simulink model "s_b2a4x1kf"  (R2018b)
settings: Solver=VariableStepDiscrete  StartTime=0.0  StopTime=100  RelTol=1e-3
undefined symbols (not defined in the file): fft_stages, n_bits_ants, n_bits_xengs
libraries: xbsIndex_r4 x20671, casper_library_misc x69, casper_library_scopes x15, casper_library_delays x8, xbsReplacements_r4 x6, xps_library x4
(part 2 of 212)

== system s_b2a4x1kf/Delay10 ==
  d : Inport
  Register0 : xbsIndex_r4/Register  init=0  rst=off  en=off  dbl_ovrd=off  block_type=register
      settings: block_version=11.4
  Register1 : xbsIndex_r4/Register  init=0  rst=off  en=off  dbl_ovrd=off  block_type=register
      settings: block_version=11.4
  q : Outport
  wires:
  Register0/1 -> Register1/1
  d/1 -> Register0/1
  Register1/1 -> q/1

== system s_b2a4x1kf/Delay16 ==
  d : Inport
  Register0 : xbsIndex_r4/Register  init=0  rst=off  en=off  dbl_ovrd=off  block_type=register
      settings: block_version=11.4
  Register1 : xbsIndex_r4/Register  init=0  rst=off  en=off  dbl_ovrd=off  block_type=register
      settings: block_version=11.4
  q : Outport
  wires:
  Register0/1 -> Register1/1
  d/1 -> Register0/1
  Register1/1 -> q/1

== system s_b2a4x1kf/Delay18 ==
  d : Inport
  Register0 : xbsIndex_r4/Register  init=0  rst=off  en=off  dbl_ovrd=off  block_type=register
      settings: block_version=11.4
  Register1 : xbsIndex_r4/Register  init=0  rst=off  en=off  dbl_ovrd=off  block_type=register
      settings: block_version=11.4
  q : Outport
  wires:
  Register0/1 -> Register1/1
  d/1 -> Register0/1
  Register1/1 -> q/1

== system s_b2a4x1kf/Delay19 ==
  d : Inport
  Register0 : xbsIndex_r4/Register  init=0  rst=off  en=off  dbl_ovrd=off  block_type=register
      settings: block_version=11.4
  Register1 : xbsIndex_r4/Register  init=0  rst=off  en=off  dbl_ovrd=off  block_type=register
      settings: block_version=11.4
  q : Outport
  wires:
  Register0/1 -> Register1/1
  d/1 -> Register0/1
  Register1/1 -> q/1

== system s_b2a4x1kf/Delay20 ==
  d : Inport
  Register0 : xbsIndex_r4/Register  init=0  rst=off  en=off  dbl_ovrd=off  block_type=register
      settings: block_version=11.4
  Register1 : xbsIndex_r4/Register  init=0  rst=off  en=off  dbl_ovrd=off  block_type=register
      settings: block_version=11.4
  q : Outport
  wires:
  Register0/1 -> Register1/1
  d/1 -> Register0/1
  Register1/1 -> q/1

== system s_b2a4x1kf/Delay21 ==
  d : Inport
  Register0 : xbsIndex_r4/Register  init=0  rst=off  en=off  dbl_ovrd=off  block_type=register
      settings: block_version=11.4
  Register1 : xbsIndex_r4/Register  init=0  rst=off  en=off  dbl_ovrd=off  block_type=register
      settings: block_version=11.4
  q : Outport
  wires:
  Register0/1 -> Register1/1
  d/1 -> Register0/1
  Register1/1 -> q/1

== system s_b2a4x1kf/Delay26 ==
  d : Inport
  Register0 : xbsIndex_r4/Register  init=0  rst=off  en=off  dbl_ovrd=off  block_type=register
      settings: block_version=11.4
  Register1 : xbsIndex_r4/Register  init=0  rst=off  en=off  dbl_ovrd=off  block_type=register
      settings: block_version=11.4
  q : Outport
  wires:
  Register0/1 -> Register1/1
  d/1 -> Register0/1
  Register1/1 -> q/1

== system s_b2a4x1kf/Delay27 ==
  d : Inport
  Register0 : xbsIndex_r4/Register  init=0  rst=off  en=off  dbl_ovrd=off  block_type=register
      settings: block_version=11.4
  Register1 : xbsIndex_r4/Register  init=0  rst=off  en=off  dbl_ovrd=off  block_type=register
      settings: block_version=11.4
  q : Outport
  wires:
  Register0/1 -> Register1/1
  d/1 -> Register0/1
  Register1/1 -> q/1

== system s_b2a4x1kf/Delay28 ==
  d : Inport
  Register0 : xbsIndex_r4/Register  init=0  rst=off  en=off  dbl_ovrd=off  block_type=register
      settings: block_version=11.4
  Register1 : xbsIndex_r4/Register  init=0  rst=off  en=off  dbl_ovrd=off  block_type=register
      settings: block_version=11.4
  q : Outport
  wires:
  Register0/1 -> Register1/1
  d/1 -> Register0/1
  Register1/1 -> q/1

== system s_b2a4x1kf/Delay32 ==
  d : Inport
  Register0 : xbsIndex_r4/Register  init=0  rst=off  en=off  dbl_ovrd=off  block_type=register
      settings: block_version=11.4
  Register1 : xbsIndex_r4/Register  init=0  rst=off  en=off  dbl_ovrd=off  block_type=register
      settings: block_version=11.4
  q : Outport
  wires:
  Register0/1 -> Register1/1
  d/1 -> Register0/1
  Register1/1 -> q/1

== system s_b2a4x1kf/Delay72 ==
  d : Inport
  Register0 : xbsIndex_r4/Register  init=0  rst=off  en=off  dbl_ovrd=off  block_type=register
      settings: block_version=11.4
  Register1 : xbsIndex_r4/Register  init=0  rst=off  en=off  dbl_ovrd=off  block_type=register
      settings: block_version=11.4
  q : Outport
  wires:
  Register0/1 -> Register1/1
  d/1 -> Register0/1
  Register1/1 -> q/1

== system s_b2a4x1kf/Delay9 ==
  d : Inport
  Register0 : xbsIndex_r4/Register  init=0  rst=off  en=off  dbl_ovrd=off  block_type=register
      settings: block_version=11.4
  Register1 : xbsIndex_r4/Register  init=0  rst=off  en=off  dbl_ovrd=off  block_type=register
      settings: block_version=11.4
  q : Outport
  wires:
  Register0/1 -> Register1/1
  d/1 -> Register0/1
  Register1/1 -> q/1

== system s_b2a4x1kf/Subsystem11 ==
  rst : Inport
  eof : Inport  Port=2
  valid : Inport  Port=3
  Counter11 : xbsIndex_r4/Counter  cnt_type=Free Running  cnt_to=Inf  operation=Up  start_count=0  cnt_by_val=1  arith_type=Unsigned  n_bits=n_bits_count  bin_pt=0  load_pin=off  rst=on  en=on  explicit_period=on  period=1  use_behavioral_HDL=off  implementation=Fabric  dbl_ovrd=off  block_type=counter
  Delay : xbsIndex_r4/Delay  rst=off  infoeditControl=Selection of Reset will increase slice count due to use of real FFs and instead of SRLs  en=off  latency=1  reg_retiming=on  dbl_ovrd=off  block_type=delay
      settings: infoedit=Hardware notes: A delay line is a chain, each link of which is an SRL16 or SRL32 followed by a flip-flop.
  Delay1 : xbsIndex_r4/Delay  rst=off  infoeditControl=Selection of Reset will increase slice count due to use of real FFs and instead of SRLs  en=off  latency=1  reg_retiming=on  dbl_ovrd=off  block_type=delay
      settings: infoedit=Hardware notes: A delay line is a chain, each link of which is an SRL16 or SRL32 followed by a flip-flop.
  Delay2 : xbsIndex_r4/Delay  rst=off  infoeditControl=Selection of Reset will increase slice count due to use of real FFs and instead of SRLs  en=off  latency=1  reg_retiming=on  dbl_ovrd=off  block_type=delay
      settings: infoedit=Hardware notes: A delay line is a chain, each link of which is an SRL16 or SRL32 followed by a flip-flop.
  Logical6 : xbsIndex_r4/Logical  logical_function=AND  inputs=2  en=off  latency=0  precision=Full  arith_type=Unsigned  n_bits=16  bin_pt=0  align_bp=on  dbl_ovrd=off  block_type=logical
  pipeline : Subsystem  Tag=cmac_delinked  mask(pipeline){csp_latency=2}
      mask prompts: csp_latency "Latency"
      mask help:
      | An explicitly laid-out delay line to avoid mapping to SRL16s
      | for use in pipelining to help achieve timing closure.
      mask init:
      | pipeline_init(gcb,'latency',csp_latency);
      settings: AttributesFormatString=Latency = %<latency>
      mask Display:
      | port_label('input', 1, 'd');
      | port_label('output', 1, 'q');
      | disp(['Z^-', num2str(csp_latency)]);
  out0 : Outport
  wires:
  pipeline/1(q) -> out0/1
  eof/1 -> Delay1/1
  Logical6/1 -> Counter11/2
  rst/1 -> Delay/1
  Delay/1 -> Counter11/1
  Counter11/1 -> pipeline/1(d)
  valid/1 -> Delay2/1
  Delay1/1 -> Logical6/1
  Delay2/1 -> Logical6/2

== system s_b2a4x1kf/Subsystem2 ==
  rst : Inport
  in0 : Inport  Port=2
  in1 : Inport  Port=3
  in2 : Inport  Port=4
  in3 : Inport  Port=5
  Counter{1..3,11} (4 alike) : xbsIndex_r4/Counter  cnt_type=Free Running  cnt_to=Inf  operation=Up  start_count=0  cnt_by_val=1  arith_type=Unsigned  n_bits=n_bits_count  bin_pt=0  load_pin=off  rst=on  en=on  explicit_period=on  period=1  use_behavioral_HDL=off  implementation=Fabric  dbl_ovrd=off  block_type=counter
  Delay{,1..4,15,17,59,61..63,76} (12 alike) : xbsIndex_r4/Delay  rst=off  infoeditControl=Selection of Reset will increase slice count due to use of real FFs and instead of SRLs  en=off  latency=1  reg_retiming=on  dbl_ovrd=off  block_type=delay
      settings: infoedit=Hardware notes: A delay line is a chain, each link of which is an SRL16 or SRL32 followed by a flip-flop.
  pipeline : Subsystem  Tag=cmac_delinked  mask(pipeline){csp_latency=2}
      mask prompts: csp_latency "Latency"
      mask help:
      | An explicitly laid-out delay line to avoid mapping to SRL16s
      | for use in pipelining to help achieve timing closure.
      mask init:
      | pipeline_init(gcb,'latency',csp_latency);
      settings: AttributesFormatString=Latency = %<latency>
      mask Display:
      | port_label('input', 1, 'd');
      | port_label('output', 1, 'q');
      | disp(['Z^-', num2str(csp_latency)]);
  pipeline1 : Subsystem  Tag=cmac_delinked  mask(pipeline){csp_latency=2}
      mask prompts: csp_latency "Latency"
      mask help:
      | An explicitly laid-out delay line to avoid mapping to SRL16s
      | for use in pipelining to help achieve timing closure.
      mask init:
      | pipeline_init(gcb,'latency',csp_latency);
      settings: AttributesFormatString=Latency = %<latency>
      mask Display:
      | port_label('input', 1, 'd');
      | port_label('output', 1, 'q');
      | disp(['Z^-', num2str(csp_latency)]);
  pipeline2 : Subsystem  Tag=cmac_delinked  mask(pipeline){csp_latency=2}
      mask prompts: csp_latency "Latency"
      mask help:
      | An explicitly laid-out delay line to avoid mapping to SRL16s
      | for use in pipelining to help achieve timing closure.
      mask init:
      | pipeline_init(gcb,'latency',csp_latency);
      settings: AttributesFormatString=Latency = %<latency>
      mask Display:
      | port_label('input', 1, 'd');
      | port_label('output', 1, 'q');
      | disp(['Z^-', num2str(csp_latency)]);
  pipeline3 : Subsystem  Tag=cmac_delinked  mask(pipeline){csp_latency=2}
      mask prompts: csp_latency "Latency"
      mask help:
      | An explicitly laid-out delay line to avoid mapping to SRL16s
      | for use in pipelining to help achieve timing closure.
      mask init:
      | pipeline_init(gcb,'latency',csp_latency);
      settings: AttributesFormatString=Latency = %<latency>
      mask Display:
      | port_label('input', 1, 'd');
      | port_label('output', 1, 'q');
      | disp(['Z^-', num2str(csp_latency)]);
  out0 : Outport
  out1 : Outport  Port=2
  out2 : Outport  Port=3
  out3 : Outport  Port=4
  wires:
  Counter11/1 -> pipeline/1(d)
  Counter1/1 -> pipeline1/1(d)
  Counter3/1 -> pipeline2/1(d)
  Delay17/1 -> Delay63/1
  Delay3/1 -> Delay62/1
  Delay15/1 -> Delay61/1
  Delay/1 -> Delay76/1, Counter11/1
  rst/1 -> Delay/1
  Delay61/1 -> Counter11/2
  Delay62/1 -> Counter1/2
  Delay63/1 -> Counter3/2
  Delay76/1 -> Counter1/1, Delay59/1
  in0/1 -> Delay15/1
  in1/1 -> Delay3/1
  in2/1 -> Delay17/1
  pipeline/1(q) -> out0/1
  pipeline1/1(q) -> out1/1
  pipeline2/1(q) -> out2/1
  Counter2/1 -> pipeline3/1(d)
  Delay1/1 -> Delay4/1
  Delay4/1 -> Counter2/2
  Delay59/1 -> Delay2/1, Counter3/1
  in3/1 -> Delay1/1
  pipeline3/1(q) -> out3/1
  Delay2/1 -> Counter2/1

== system s_b2a4x1kf/Subsystem7 ==
  dv : Inport
  Constant8 : xbsIndex_r4/Constant  const=clk_rate  gui_display_data_type=Fixed-point  arith_type=Unsigned  n_bits=ceil(log2(clk_rate))  bin_pt=0  preci_type=Single  exp_width=8  frac_width=24  explicit_period=on  period=1  equ=P=C  opselect=C  inp2=PCIN>>17  opr=+  inp1=P  carry=CIN  dbl_ovrd=off  block_type=constant
      settings: block_version=11.4
  Counter1 : xbsIndex_r4/Counter  cnt_type=Count Limited  cnt_to=clk_rate  operation=Up  start_count=0  cnt_by_val=1  arith_type=Unsigned  n_bits=ceil(log2(clk_rate))  bin_pt=0  load_pin=off  rst=off  en=off  explicit_period=on  period=1  use_behavioral_HDL=off  implementation=Fabric  dbl_ovrd=off  block_type=counter
  Counter6 : xbsIndex_r4/Counter  cnt_type=Free Running  cnt_to=Inf  operation=Up  start_count=0  cnt_by_val=1  arith_type=Unsigned  n_bits=32  bin_pt=0  load_pin=off  rst=on  en=on  explicit_period=on  period=1  use_behavioral_HDL=off  implementation=Fabric  dbl_ovrd=off  block_type=counter
  Delay : xbsIndex_r4/Delay  rst=off  infoeditControl=Selection of Reset will increase slice count due to use of real FFs and instead of SRLs  en=on  latency=1  reg_retiming=on  dbl_ovrd=off  block_type=delay
      settings: infoedit=Hardware notes: A delay line is a chain, each link of which is an SRL16 or SRL32 followed by a flip-flop.
  Delay5 : xbsIndex_r4/Delay  rst=off  infoeditControl=Selection of Reset will increase slice count due to use of real FFs and instead of SRLs  en=off  latency=1  reg_retiming=on  dbl_ovrd=off  block_type=delay
      settings: infoedit=Hardware notes: A delay line is a chain, each link of which is an SRL16 or SRL32 followed by a flip-flop.
  Relational : xbsIndex_r4/Relational  mode=a=b  op_type=Bool  en=off  latency=1  dbl_ovrd=off  block_type=relational
  per_sec : Outport
  wires:
  Delay/1 -> per_sec/1
  Counter6/1 -> Delay/1
  dv/1 -> Delay5/1
  Relational/1 -> Delay/2, Counter6/1
  Counter1/1 -> Relational/1
  Delay5/1 -> Counter6/2
  Constant8/1 -> Relational/2

== system s_b2a4x1kf/acc_len ==
  convert1_1 : DataTypeConversion  OutDataTypeStr=fixdt('ufix32_En0')  LockScale=on
  convert2_1 : DataTypeConversion  OutDataTypeStr=fixdt('ufix32_En0')  ConvertRealWorld=Stored Integer (SI)  LockScale=on
  gain_1 : Gain
  io_delay : xbsIndex_r4/Delay  rst=off  infoeditControl=Selection of Reset will increase slice count due to use of real FFs and instead of SRLs  en=off  latency=0  reg_retiming=on  dbl_ovrd=off  block_type=delay
  reint1 : xbsIndex_r4/Reinterpret  force_arith_type=on  arith_type=Unsigned  force_bin_pt=on  bin_pt=0  block_type=reinterpret
  s_b2a4x1kf_acc_len_user_data_out : xbsIndex_r4/Gateway In  gui_display_data_type=Fixed-point  arith_type=Unsigned  n_bits=32  bin_pt=0  preci_type=Single  exp_width=8  frac_width=24  rows=1  columns=1  quantization="Round  (unbiased: +/- Inf)"  overflow=Saturate  period=1  UseAsADC=off  ADCChannel='1'  interface=None  automatic_assignment=on  address_offset=hex2dec('00')  intf_name=''  intf_description=''  default_value=0  timing_constraint=None  locs_specified=off  LOCs={}  io_standard={}  inherit_from_input=off  hdl_port=on  dbl_ovrd=off  block_type=gatewayin
  sim_1 : Constant  Value=0
  slice_reg : xbsIndex_r4/Slice  nbits=32  boolean_output=off  mode=Lower Bit Location + Width  bit1=0  base1=MSB of Input  bit0=0  base0=LSB of Input  dbl_ovrd=off  block_type=slice
  in_reg : Outport
  wires:
  s_b2a4x1kf_acc_len_user_data_out/1 -> io_delay/1
  sim_1/1 -> convert1_1/1
  convert1_1/1 -> convert2_1/1
  convert2_1/1 -> gain_1/1
  gain_1/1 -> s_b2a4x1kf_acc_len_user_data_out/1
  io_delay/1 -> slice_reg/1
  slice_reg/1 -> reint1/1
  reint1/1 -> in_reg/1

== system s_b2a4x1kf/bf0_config ==
  convert1_1 : DataTypeConversion  OutDataTypeStr=fixdt('ufix15_En8')  LockScale=on
  convert1_2 : DataTypeConversion  OutDataTypeStr=fixdt('ufix16_En0')  LockScale=on
  convert1_3 : DataTypeConversion  OutDataTypeStr=fixdt('ufix1_En0')  LockScale=on
  convert2_1 : DataTypeConversion  OutDataTypeStr=fixdt('ufix15_En0')  ConvertRealWorld=Stored Integer (SI)  LockScale=on
  convert2_2 : DataTypeConversion  OutDataTypeStr=fixdt('ufix16_En0')  ConvertRealWorld=Stored Integer (SI)  LockScale=on
  convert2_3 : DataTypeConversion  OutDataTypeStr=fixdt('ufix1_En0')  ConvertRealWorld=Stored Integer (SI)  LockScale=on
  gain_1 : Gain  Gain=131072
  gain_2 : Gain  Gain=2
  gain_3 : Gain
  io_delay : xbsIndex_r4/Delay  rst=off  infoeditControl=Selection of Reset will increase slice count due to use of real FFs and instead of SRLs  en=off  latency=0  reg_retiming=on  dbl_ovrd=off  block_type=delay
  reint1 : xbsIndex_r4/Reinterpret  force_arith_type=on  arith_type=Unsigned  force_bin_pt=on  bin_pt=8  block_type=reinterpret
  reint2 : xbsIndex_r4/Reinterpret  force_arith_type=on  arith_type=Unsigned  force_bin_pt=on  bin_pt=0  block_type=reinterpret
  s_b2a4x1kf_bf0_config_user_data_out : xbsIndex_r4/Gateway In  gui_display_data_type=Fixed-point  arith_type=Unsigned  n_bits=32  bin_pt=0  preci_type=Single  exp_width=8  frac_width=24  rows=1  columns=1  quantization="Round  (unbiased: +/- Inf)"  overflow=Saturate  period=1  UseAsADC=off  ADCChannel='1'  interface=None  automatic_assignment=on  address_offset=hex2dec('00')  intf_name=''  intf_description=''  default_value=0  timing_constraint=None  locs_specified=off  LOCs={}  io_standard={}  inherit_from_input=off  hdl_port=on  dbl_ovrd=off  block_type=gatewayin
  sim_1 : Constant  Value=0
  sim_2 : Constant  Value=0
  sim_3 : Constant  Value=0
  sim_add : Sum  Inputs=+++  OutDataTypeStr=uint32
  slice_port : xbsIndex_r4/Slice  nbits=16  boolean_output=off  mode=Lower Bit Location + Width  bit1=0  base1=MSB of Input  bit0=1  base0=LSB of Input  dbl_ovrd=off  block_type=slice
  slice_quant_gain : xbsIndex_r4/Slice  nbits=15  boolean_output=off  mode=Lower Bit Location + Width  bit1=0  base1=MSB of Input  bit0=17  base0=LSB of Input  dbl_ovrd=off  block_type=slice
  slice_txen : xbsIndex_r4/Slice  nbits=1  boolean_output=on  mode=Lower Bit Location + Width  bit1=0  base1=MSB of Input  bit0=0  base0=LSB of Input  dbl_ovrd=off  block_type=slice
  in_quant_gain : Outport
  in_port : Outport  Port=2
  in_txen : Outport  Port=3
  wires:
  s_b2a4x1kf_bf0_config_user_data_out/1 -> io_delay/1
  sim_add/1 -> s_b2a4x1kf_bf0_config_user_data_out/1
  sim_1/1 -> convert1_1/1
  convert1_1/1 -> convert2_1/1
  convert2_1/1 -> gain_1/1
  gain_1/1 -> sim_add/1
  io_delay/1 -> slice_quant_gain/1, slice_port/1, slice_txen/1
  slice_quant_gain/1 -> reint1/1
  reint1/1 -> in_quant_gain/1
  sim_2/1 -> convert1_2/1
  convert1_2/1 -> convert2_2/1
  convert2_2/1 -> gain_2/1
  gain_2/1 -> sim_add/2
  slice_port/1 -> reint2/1
  reint2/1 -> in_port/1
  sim_3/1 -> convert1_3/1
  convert1_3/1 -> convert2_3/1
  convert2_3/1 -> gain_3/1
  gain_3/1 -> sim_add/3
  slice_txen/1 -> in_txen/1

== system s_b2a4x1kf/bf0_ip ==
  convert1_1 : DataTypeConversion  OutDataTypeStr=fixdt('ufix32_En0')  LockScale=on
  convert2_1 : DataTypeConversion  OutDataTypeStr=fixdt('ufix32_En0')  ConvertRealWorld=Stored Integer (SI)  LockScale=on
  gain_1 : Gain
  io_delay : xbsIndex_r4/Delay  rst=off  infoeditControl=Selection of Reset will increase slice count due to use of real FFs and instead of SRLs  en=off  latency=0  reg_retiming=on  dbl_ovrd=off  block_type=delay
  reint1 : xbsIndex_r4/Reinterpret  force_arith_type=on  arith_type=Unsigned  force_bin_pt=on  bin_pt=0  block_type=reinterpret
  s_b2a4x1kf_bf0_ip_user_data_out : xbsIndex_r4/Gateway In  gui_display_data_type=Fixed-point  arith_type=Unsigned  n_bits=32  bin_pt=0  preci_type=Single  exp_width=8  frac_width=24  rows=1  columns=1  quantization="Round  (unbiased: +/- Inf)"  overflow=Saturate  period=1  UseAsADC=off  ADCChannel='1'  interface=None  automatic_assignment=on  address_offset=hex2dec('00')  intf_name=''  intf_description=''  default_value=0  timing_constraint=None  locs_specified=off  LOCs={}  io_standard={}  inherit_from_input=off  hdl_port=on  dbl_ovrd=off  block_type=gatewayin
  sim_1 : Constant  Value=0
  slice_ip : xbsIndex_r4/Slice  nbits=32  boolean_output=off  mode=Lower Bit Location + Width  bit1=0  base1=MSB of Input  bit0=0  base0=LSB of Input  dbl_ovrd=off  block_type=slice
  in_ip : Outport
  wires:
  s_b2a4x1kf_bf0_ip_user_data_out/1 -> io_delay/1
  sim_1/1 -> convert1_1/1
  convert1_1/1 -> convert2_1/1
  convert2_1/1 -> gain_1/1
  gain_1/1 -> s_b2a4x1kf_bf0_ip_user_data_out/1
  io_delay/1 -> slice_ip/1
  slice_ip/1 -> reint1/1
  reint1/1 -> in_ip/1

== system s_b2a4x1kf/bf1_config ==
  convert1_1 : DataTypeConversion  OutDataTypeStr=fixdt('ufix15_En8')  LockScale=on
  convert1_2 : DataTypeConversion  OutDataTypeStr=fixdt('ufix16_En0')  LockScale=on
  convert1_3 : DataTypeConversion  OutDataTypeStr=fixdt('ufix1_En0')  LockScale=on
  convert2_1 : DataTypeConversion  OutDataTypeStr=fixdt('ufix15_En0')  ConvertRealWorld=Stored Integer (SI)  LockScale=on
  convert2_2 : DataTypeConversion  OutDataTypeStr=fixdt('ufix16_En0')  ConvertRealWorld=Stored Integer (SI)  LockScale=on
  convert2_3 : DataTypeConversion  OutDataTypeStr=fixdt('ufix1_En0')  ConvertRealWorld=Stored Integer (SI)  LockScale=on
  gain_1 : Gain  Gain=131072
  gain_2 : Gain  Gain=2
  gain_3 : Gain
  io_delay : xbsIndex_r4/Delay  rst=off  infoeditControl=Selection of Reset will increase slice count due to use of real FFs and instead of SRLs  en=off  latency=0  reg_retiming=on  dbl_ovrd=off  block_type=delay
  reint1 : xbsIndex_r4/Reinterpret  force_arith_type=on  arith_type=Unsigned  force_bin_pt=on  bin_pt=8  block_type=reinterpret
  reint2 : xbsIndex_r4/Reinterpret  force_arith_type=on  arith_type=Unsigned  force_bin_pt=on  bin_pt=0  block_type=reinterpret
  s_b2a4x1kf_bf1_config_user_data_out : xbsIndex_r4/Gateway In  gui_display_data_type=Fixed-point  arith_type=Unsigned  n_bits=32  bin_pt=0  preci_type=Single  exp_width=8  frac_width=24  rows=1  columns=1  quantization="Round  (unbiased: +/- Inf)"  overflow=Saturate  period=1  UseAsADC=off  ADCChannel='1'  interface=None  automatic_assignment=on  address_offset=hex2dec('00')  intf_name=''  intf_description=''  default_value=0  timing_constraint=None  locs_specified=off  LOCs={}  io_standard={}  inherit_from_input=off  hdl_port=on  dbl_ovrd=off  block_type=gatewayin
  sim_1 : Constant  Value=0
  sim_2 : Constant  Value=0
  sim_3 : Constant  Value=0
  sim_add : Sum  Inputs=+++  OutDataTypeStr=uint32
  slice_port : xbsIndex_r4/Slice  nbits=16  boolean_output=off  mode=Lower Bit Location + Width  bit1=0  base1=MSB of Input  bit0=1  base0=LSB of Input  dbl_ovrd=off  block_type=slice
  slice_quant_gain : xbsIndex_r4/Slice  nbits=15  boolean_output=off  mode=Lower Bit Location + Width  bit1=0  base1=MSB of Input  bit0=17  base0=LSB of Input  dbl_ovrd=off  block_type=slice
  slice_txen : xbsIndex_r4/Slice  nbits=1  boolean_output=on  mode=Lower Bit Location + Width  bit1=0  base1=MSB of Input  bit0=0  base0=LSB of Input  dbl_ovrd=off  block_type=slice
  in_quant_gain : Outport
  in_port : Outport  Port=2
  in_txen : Outport  Port=3
  wires:
  s_b2a4x1kf_bf1_config_user_data_out/1 -> io_delay/1
  sim_add/1 -> s_b2a4x1kf_bf1_config_user_data_out/1
  sim_1/1 -> convert1_1/1
  convert1_1/1 -> convert2_1/1
  convert2_1/1 -> gain_1/1
  gain_1/1 -> sim_add/1
  io_delay/1 -> slice_quant_gain/1, slice_port/1, slice_txen/1
  slice_quant_gain/1 -> reint1/1
  reint1/1 -> in_quant_gain/1
  sim_2/1 -> convert1_2/1
  convert1_2/1 -> convert2_2/1
  convert2_2/1 -> gain_2/1
  gain_2/1 -> sim_add/2
  slice_port/1 -> reint2/1
  reint2/1 -> in_port/1
  sim_3/1 -> convert1_3/1
  convert1_3/1 -> convert2_3/1
  convert2_3/1 -> gain_3/1
  gain_3/1 -> sim_add/3
  slice_txen/1 -> in_txen/1

== system s_b2a4x1kf/bf1_ip ==
  convert1_1 : DataTypeConversion  OutDataTypeStr=fixdt('ufix32_En0')  LockScale=on
  convert2_1 : DataTypeConversion  OutDataTypeStr=fixdt('ufix32_En0')  ConvertRealWorld=Stored Integer (SI)  LockScale=on
  gain_1 : Gain
  io_delay : xbsIndex_r4/Delay  rst=off  infoeditControl=Selection of Reset will increase slice count due to use of real FFs and instead of SRLs  en=off  latency=0  reg_retiming=on  dbl_ovrd=off  block_type=delay
  reint1 : xbsIndex_r4/Reinterpret  force_arith_type=on  arith_type=Unsigned  force_bin_pt=on  bin_pt=0  block_type=reinterpret
  s_b2a4x1kf_bf1_ip_user_data_out : xbsIndex_r4/Gateway In  gui_display_data_type=Fixed-point  arith_type=Unsigned  n_bits=32  bin_pt=0  preci_type=Single  exp_width=8  frac_width=24  rows=1  columns=1  quantization="Round  (unbiased: +/- Inf)"  overflow=Saturate  period=1  UseAsADC=off  ADCChannel='1'  interface=None  automatic_assignment=on  address_offset=hex2dec('00')  intf_name=''  intf_description=''  default_value=0  timing_constraint=None  locs_specified=off  LOCs={}  io_standard={}  inherit_from_input=off  hdl_port=on  dbl_ovrd=off  block_type=gatewayin
  sim_1 : Constant  Value=0
  slice_ip : xbsIndex_r4/Slice  nbits=32  boolean_output=off  mode=Lower Bit Location + Width  bit1=0  base1=MSB of Input  bit0=0  base0=LSB of Input  dbl_ovrd=off  block_type=slice
  in_ip : Outport
  wires:
  s_b2a4x1kf_bf1_ip_user_data_out/1 -> io_delay/1
  sim_1/1 -> convert1_1/1
  convert1_1/1 -> convert2_1/1
  convert2_1/1 -> gain_1/1
  gain_1/1 -> s_b2a4x1kf_bf1_ip_user_data_out/1
  io_delay/1 -> slice_ip/1
  slice_ip/1 -> reint1/1
  reint1/1 -> in_ip/1

== system s_b2a4x1kf/bf_config ==
  convert1_1 : DataTypeConversion  OutDataTypeStr=fixdt('ufix8_En0')  LockScale=on
  convert1_2 : DataTypeConversion  OutDataTypeStr=fixdt('ufix16_En0')  LockScale=on
  convert1_3 : DataTypeConversion  OutDataTypeStr=fixdt('ufix1_En0')  LockScale=on
  convert1_4 : DataTypeConversion  OutDataTypeStr=fixdt('ufix1_En0')  LockScale=on
  convert1_5 : DataTypeConversion  OutDataTypeStr=fixdt('ufix1_En0')  LockScale=on
  convert2_1 : DataTypeConversion  OutDataTypeStr=fixdt('ufix8_En0')  ConvertRealWorld=Stored Integer (SI)  LockScale=on
  convert2_2 : DataTypeConversion  OutDataTypeStr=fixdt('ufix16_En0')  ConvertRealWorld=Stored Integer (SI)  LockScale=on
  convert2_3 : DataTypeConversion  OutDataTypeStr=fixdt('ufix1_En0')  ConvertRealWorld=Stored Integer (SI)  LockScale=on
  convert2_4 : DataTypeConversion  OutDataTypeStr=fixdt('ufix1_En0')  ConvertRealWorld=Stored Integer (SI)  LockScale=on
  convert2_5 : DataTypeConversion  OutDataTypeStr=fixdt('ufix1_En0')  ConvertRealWorld=Stored Integer (SI)  LockScale=on
  gain_1 : Gain  Gain=524288
  gain_2 : Gain  Gain=8
  gain_3 : Gain  Gain=4
  gain_4 : Gain  Gain=2
  gain_5 : Gain
  io_delay : xbsIndex_r4/Delay  rst=off  infoeditControl=Selection of Reset will increase slice count due to use of real FFs and instead of SRLs  en=off  latency=0  reg_retiming=on  dbl_ovrd=off  block_type=delay
  reint1 : xbsIndex_r4/Reinterpret  force_arith_type=on  arith_type=Unsigned  force_bin_pt=on  bin_pt=0  block_type=reinterpret
  reint2 : xbsIndex_r4/Reinterpret  force_arith_type=on  arith_type=Unsigned  force_bin_pt=on  bin_pt=0  block_type=reinterpret
  s_b2a4x1kf_bf_config_user_data_out : xbsIndex_r4/Gateway In  gui_display_data_type=Fixed-point  arith_type=Unsigned  n_bits=32  bin_pt=0  preci_type=Single  exp_width=8  frac_width=24  rows=1  columns=1  quantization="Round  (unbiased: +/- Inf)"  overflow=Saturate  period=1  UseAsADC=off  ADCChannel='1'  interface=None  automatic_assignment=on  address_offset=hex2dec('00')  intf_name=''  intf_description=''  default_value=0  timing_constraint=None  locs_specified=off  LOCs={}  io_standard={}  inherit_from_input=off  hdl_port=on  dbl_ovrd=off  block_type=gatewayin
  sim_{1..5} (5 alike) : Constant  Value=0
  sim_add : Sum  Inputs=+++++  OutDataTypeStr=uint32
  slice_data_id : xbsIndex_r4/Slice  nbits=8  boolean_output=off  mode=Lower Bit Location + Width  bit1=0  base1=MSB of Input  bit0=19  base0=LSB of Input  dbl_ovrd=off  block_type=slice
  slice_snap_arm : xbsIndex_r4/Slice  nbits=1  boolean_output=on  mode=Lower Bit Location + Width  bit1=0  base1=MSB of Input  bit0=1  base0=LSB of Input  dbl_ovrd=off  block_type=slice
  slice_snap_trig : xbsIndex_r4/Slice  nbits=1  boolean_output=on  mode=Lower Bit Location + Width  bit1=0  base1=MSB of Input  bit0=0  base0=LSB of Input  dbl_ovrd=off  block_type=slice
  slice_time_id : xbsIndex_r4/Slice  nbits=16  boolean_output=off  mode=Lower Bit Location + Width  bit1=0  base1=MSB of Input  bit0=3  base0=LSB of Input  dbl_ovrd=off  block_type=slice
  slice_tvg_sel : xbsIndex_r4/Slice  nbits=1  boolean_output=on  mode=Lower Bit Location + Width  bit1=0  base1=MSB of Input  bit0=2  base0=LSB of Input  dbl_ovrd=off  block_type=slice
  in_data_id : Outport
  in_time_id : Outport  Port=2
  in_tvg_sel : Outport  Port=3
  in_snap_arm : Outport  Port=4
  in_snap_trig : Outport  Port=5
  wires:
  s_b2a4x1kf_bf_config_user_data_out/1 -> io_delay/1
  sim_add/1 -> s_b2a4x1kf_bf_config_user_data_out/1
  sim_1/1 -> convert1_1/1
  convert1_1/1 -> convert2_1/1
  convert2_1/1 -> gain_1/1
  gain_1/1 -> sim_add/1
  io_delay/1 -> slice_data_id/1, slice_time_id/1, slice_tvg_sel/1, slice_snap_arm/1, slice_snap_trig/1
  slice_data_id/1 -> reint1/1
  reint1/1 -> in_data_id/1
  sim_2/1 -> convert1_2/1
  convert1_2/1 -> convert2_2/1
  convert2_2/1 -> gain_2/1
  gain_2/1 -> sim_add/2
  slice_time_id/1 -> reint2/1
  reint2/1 -> in_time_id/1
  sim_3/1 -> convert1_3/1
  convert1_3/1 -> convert2_3/1
  convert2_3/1 -> gain_3/1
  gain_3/1 -> sim_add/3
  slice_tvg_sel/1 -> in_tvg_sel/1
  sim_4/1 -> convert1_4/1
  convert1_4/1 -> convert2_4/1
  convert2_4/1 -> gain_4/1
  gain_4/1 -> sim_add/4
  slice_snap_arm/1 -> in_snap_arm/1
  sim_5/1 -> convert1_5/1
  convert1_5/1 -> convert2_5/1
  convert2_5/1 -> gain_5/1
  gain_5/1 -> sim_add/5
  slice_snap_trig/1 -> in_snap_trig/1

== system s_b2a4x1kf/bf_valout_bw0 ==
  out_bw0 : Inport
  out_bw1 : Inport  Port=2
  assert_bw0 : xbsIndex_r4/Assert  assert_type=on  type_source=Explicitly  gui_display_data_type=Fixed-point  arith_type="Signed  (2's comp)"  n_bits=16  bin_pt=9  preci_type=Single  exp_width=8  frac_width=24  assert_rate=off  rate_source=Explicitly  period=1  output_port=on  block_type=assert
  assert_bw1 : xbsIndex_r4/Assert  assert_type=on  type_source=Explicitly  gui_display_data_type=Fixed-point  arith_type="Signed  (2's comp)"  n_bits=16  bin_pt=9  preci_type=Single  exp_width=8  frac_width=24  assert_rate=off  rate_source=Explicitly  period=1  output_port=on  block_type=assert
  cast_gw : xbsIndex_r4/Convert  gui_display_data_type=Fixed-point  arith_type=Unsigned  n_bits=32  bin_pt=0  float_type=Single  exp_bits=8  fraction_bits=24  quantization=Truncate  overflow=Wrap  en=off  latency=1  pipeline=off  dbl_ovrd=off  block_type=convert
  concatenate : xbsIndex_r4/Concat  num_inputs=2  dbl_ovrd=off  block_type=concat
  io_delay : xbsIndex_r4/Delay  rst=off  infoeditControl=Selection of Reset will increase slice count due to use of real FFs and instead of SRLs  en=off  latency=1  reg_retiming=on  dbl_ovrd=off  block_type=delay
  reint1 : xbsIndex_r4/Reinterpret  force_arith_type=on  arith_type=Unsigned  force_bin_pt=on  bin_pt=0  block_type=reinterpret
  reint2 : xbsIndex_r4/Reinterpret  force_arith_type=on  arith_type=Unsigned  force_bin_pt=on  bin_pt=0  block_type=reinterpret
  s_b2a4x1kf_bf_valout_bw0_user_data_in : xbsIndex_r4/Gateway Out  inherit_from_input=off  hdl_port=on  rows=1  columns=1  UseAsDAC=off  DACChannel='1'  interface=None  automatic_assignment=on  address_offset=hex2dec('00')  intf_name=''  intf_description=''  timing_constraint=None  locs_specified=off  LOCs={}  io_standard={}  block_type=gatewayout
  sim_out : Terminator
  wires:
  concatenate/1 -> io_delay/1
  io_delay/1 -> cast_gw/1
  cast_gw/1 -> s_b2a4x1kf_bf_valout_bw0_user_data_in/1
  s_b2a4x1kf_bf_valout_bw0_user_data_in/1 -> sim_out/1
  out_bw0/1 -> assert_bw0/1
  assert_bw0/1 -> reint1/1
  reint1/1 -> concatenate/1
  out_bw1/1 -> assert_bw1/1
  assert_bw1/1 -> reint2/1
  reint2/1 -> concatenate/2

== system s_b2a4x1kf/bf_valout_bw1 ==
  out_bw2 : Inport
  out_bw3 : Inport  Port=2
  assert_bw2 : xbsIndex_r4/Assert  assert_type=on  type_source=Explicitly  gui_display_data_type=Fixed-point  arith_type="Signed  (2's comp)"  n_bits=16  bin_pt=9  preci_type=Single  exp_width=8  frac_width=24  assert_rate=off  rate_source=Explicitly  period=1  output_port=on  block_type=assert
  assert_bw3 : xbsIndex_r4/Assert  assert_type=on  type_source=Explicitly  gui_display_data_type=Fixed-point  arith_type="Signed  (2's comp)"  n_bits=16  bin_pt=9  preci_type=Single  exp_width=8  frac_width=24  assert_rate=off  rate_source=Explicitly  period=1  output_port=on  block_type=assert
  cast_gw : xbsIndex_r4/Convert  gui_display_data_type=Fixed-point  arith_type=Unsigned  n_bits=32  bin_pt=0  float_type=Single  exp_bits=8  fraction_bits=24  quantization=Truncate  overflow=Wrap  en=off  latency=1  pipeline=off  dbl_ovrd=off  block_type=convert
  concatenate : xbsIndex_r4/Concat  num_inputs=2  dbl_ovrd=off  block_type=concat
  io_delay : xbsIndex_r4/Delay  rst=off  infoeditControl=Selection of Reset will increase slice count due to use of real FFs and instead of SRLs  en=off  latency=1  reg_retiming=on  dbl_ovrd=off  block_type=delay
  reint1 : xbsIndex_r4/Reinterpret  force_arith_type=on  arith_type=Unsigned  force_bin_pt=on  bin_pt=0  block_type=reinterpret
  reint2 : xbsIndex_r4/Reinterpret  force_arith_type=on  arith_type=Unsigned  force_bin_pt=on  bin_pt=0  block_type=reinterpret
  s_b2a4x1kf_bf_valout_bw1_user_data_in : xbsIndex_r4/Gateway Out  inherit_from_input=off  hdl_port=on  rows=1  columns=1  UseAsDAC=off  DACChannel='1'  interface=None  automatic_assignment=on  address_offset=hex2dec('00')  intf_name=''  intf_description=''  timing_constraint=None  locs_specified=off  LOCs={}  io_standard={}  block_type=gatewayout
  sim_out : Terminator
  wires:
  concatenate/1 -> io_delay/1
  io_delay/1 -> cast_gw/1
  cast_gw/1 -> s_b2a4x1kf_bf_valout_bw1_user_data_in/1
  s_b2a4x1kf_bf_valout_bw1_user_data_in/1 -> sim_out/1
  out_bw2/1 -> assert_bw2/1
  assert_bw2/1 -> reint1/1
  reint1/1 -> concatenate/1
  out_bw3/1 -> assert_bw3/1
  assert_bw3/1 -> reint2/1
  reint2/1 -> concatenate/2

== system s_b2a4x1kf/bf_weight ==
  convert1_1 : DataTypeConversion  OutDataTypeStr=fixdt('ufix1_En0')  LockScale=on
  convert1_2 : DataTypeConversion  OutDataTypeStr=fixdt('ufix1_En0')  LockScale=on
  convert1_3 : DataTypeConversion  OutDataTypeStr=fixdt('ufix1_En0')  LockScale=on
  convert1_4 : DataTypeConversion  OutDataTypeStr=fixdt('ufix16_En9')  LockScale=on
  convert2_1 : DataTypeConversion  OutDataTypeStr=fixdt('ufix1_En0')  ConvertRealWorld=Stored Integer (SI)  LockScale=on
  convert2_2 : DataTypeConversion  OutDataTypeStr=fixdt('ufix1_En0')  ConvertRealWorld=Stored Integer (SI)  LockScale=on
  convert2_3 : DataTypeConversion  OutDataTypeStr=fixdt('ufix1_En0')  ConvertRealWorld=Stored Integer (SI)  LockScale=on
  convert2_4 : DataTypeConversion  OutDataTypeStr=fixdt('ufix16_En0')  ConvertRealWorld=Stored Integer (SI)  LockScale=on
  gain_1 : Gain  Gain=262144
  gain_2 : Gain  Gain=131072
  gain_3 : Gain  Gain=65536
  gain_4 : Gain
  io_delay : xbsIndex_r4/Delay  rst=off  infoeditControl=Selection of Reset will increase slice count due to use of real FFs and instead of SRLs  en=off  latency=0  reg_retiming=on  dbl_ovrd=off  block_type=delay
  reint1 : xbsIndex_r4/Reinterpret  force_arith_type=on  arith_type=Unsigned  force_bin_pt=on  bin_pt=0  block_type=reinterpret
  reint2 : xbsIndex_r4/Reinterpret  force_arith_type=on  arith_type=Unsigned  force_bin_pt=on  bin_pt=0  block_type=reinterpret
  reint4 : xbsIndex_r4/Reinterpret  force_arith_type=on  arith_type="Signed  (2's comp)"  force_bin_pt=on  bin_pt=9  block_type=reinterpret
  s_b2a4x1kf_bf_weight_user_data_out : xbsIndex_r4/Gateway In  gui_display_data_type=Fixed-point  arith_type=Unsigned  n_bits=32  bin_pt=0  preci_type=Single  exp_width=8  frac_width=24  rows=1  columns=1  quantization="Round  (unbiased: +/- Inf)"  overflow=Saturate  period=1  UseAsADC=off  ADCChannel='1'  interface=None  automatic_assignment=on  address_offset=hex2dec('00')  intf_name=''  intf_description=''  default_value=0  timing_constraint=None  locs_specified=off  LOCs={}  io_standard={}  inherit_from_input=off  hdl_port=on  dbl_ovrd=off  block_type=gatewayin
  sim_{1..4} (4 alike) : Constant  Value=0
  sim_add : Sum  Inputs=++++  OutDataTypeStr=uint32
  slice_antenna : xbsIndex_r4/Slice  nbits=1  boolean_output=off  mode=Lower Bit Location + Width  bit1=0  base1=MSB of Input  bit0=17  base0=LSB of Input  dbl_ovrd=off  block_type=slice
  slice_load_now : xbsIndex_r4/Slice  nbits=1  boolean_output=on  mode=Lower Bit Location + Width  bit1=0  base1=MSB of Input  bit0=16  base0=LSB of Input  dbl_ovrd=off  block_type=slice
  slice_stream : xbsIndex_r4/Slice  nbits=1  boolean_output=off  mode=Lower Bit Location + Width  bit1=0  base1=MSB of Input  bit0=18  base0=LSB of Input  dbl_ovrd=off  block_type=slice
  slice_weight : xbsIndex_r4/Slice  nbits=16  boolean_output=off  mode=Lower Bit Location + Width  bit1=0  base1=MSB of Input  bit0=0  base0=LSB of Input  dbl_ovrd=off  block_type=slice
  in_stream : Outport
  in_antenna : Outport  Port=2
  in_load_now : Outport  Port=3
  in_weight : Outport  Port=4
  wires:
  s_b2a4x1kf_bf_weight_user_data_out/1 -> io_delay/1
  sim_add/1 -> s_b2a4x1kf_bf_weight_user_data_out/1
  sim_1/1 -> convert1_1/1
  convert1_1/1 -> convert2_1/1
  convert2_1/1 -> gain_1/1
  gain_1/1 -> sim_add/1
  io_delay/1 -> slice_stream/1, slice_antenna/1, slice_load_now/1, slice_weight/1
  slice_stream/1 -> reint1/1
  reint1/1 -> in_stream/1
  sim_2/1 -> convert1_2/1
  convert1_2/1 -> convert2_2/1
  convert2_2/1 -> gain_2/1
  gain_2/1 -> sim_add/2
  slice_antenna/1 -> reint2/1
  reint2/1 -> in_antenna/1
  sim_3/1 -> convert1_3/1
  convert1_3/1 -> convert2_3/1
  convert2_3/1 -> gain_3/1
  gain_3/1 -> sim_add/3
  slice_load_now/1 -> in_load_now/1
  sim_4/1 -> convert1_4/1
  convert1_4/1 -> convert2_4/1
  convert2_4/1 -> gain_4/1
  gain_4/1 -> sim_add/4
  slice_weight/1 -> reint4/1
  reint4/1 -> in_weight/1

== system s_b2a4x1kf/board_id ==
  convert1_1 : DataTypeConversion  OutDataTypeStr=fixdt('ufix32_En0')  LockScale=on
  convert2_1 : DataTypeConversion  OutDataTypeStr=fixdt('ufix32_En0')  ConvertRealWorld=Stored Integer (SI)  LockScale=on
  gain_1 : Gain
  io_delay : xbsIndex_r4/Delay  rst=off  infoeditControl=Selection of Reset will increase slice count due to use of real FFs and instead of SRLs  en=off  latency=0  reg_retiming=on  dbl_ovrd=off  block_type=delay
  reint1 : xbsIndex_r4/Reinterpret  force_arith_type=on  arith_type=Unsigned  force_bin_pt=on  bin_pt=0  block_type=reinterpret
  s_b2a4x1kf_board_id_user_data_out : xbsIndex_r4/Gateway In  gui_display_data_type=Fixed-point  arith_type=Unsigned  n_bits=32  bin_pt=0  preci_type=Single  exp_width=8  frac_width=24  rows=1  columns=1  quantization="Round  (unbiased: +/- Inf)"  overflow=Saturate  period=1  UseAsADC=off  ADCChannel='1'  interface=None  automatic_assignment=on  address_offset=hex2dec('00')  intf_name=''  intf_description=''  default_value=0  timing_constraint=None  locs_specified=off  LOCs={}  io_standard={}  inherit_from_input=off  hdl_port=on  dbl_ovrd=off  block_type=gatewayin
  sim_1 : Constant  Value=0
  slice_reg : xbsIndex_r4/Slice  nbits=32  boolean_output=off  mode=Lower Bit Location + Width  bit1=0  base1=MSB of Input  bit0=0  base0=LSB of Input  dbl_ovrd=off  block_type=slice
  in_reg : Outport
  wires:
  s_b2a4x1kf_board_id_user_data_out/1 -> io_delay/1
  sim_1/1 -> convert1_1/1
  convert1_1/1 -> convert2_1/1
  convert2_1/1 -> gain_1/1
  gain_1/1 -> s_b2a4x1kf_board_id_user_data_out/1
  io_delay/1 -> slice_reg/1
  slice_reg/1 -> reint1/1
  reint1/1 -> in_reg/1

== system s_b2a4x1kf/bus_addsub ==
  a : Inport
  b : Inport  Port=2
  a_debus : Subsystem  AncestorBlock=casper_library_flow_control/bus_expand  mask(bus_expand){mode=divisions of arbitrary size, outputNum=1, outputWidth=[32  32  32  32  32  32  32  32  32  32  32  32], outputBinaryPt=[0  0  0  0  0  0  0  0  0  0  0  0], outputArithmeticType=[0  0  0  0  0  0  0  0  0  0  0  0], show_format=on, outputToWorkspace=off, variablePrefix=, outputToModelAsWell=on}
      mask prompts: outputNum "Number of outputs:"; outputWidth "Output width [msb ... lsb]:"; outputBinaryPt "Output binary point position [msb ... lsb]:"; outputArithmeticType "Output arithmetic type (ufix=0, fix=1, bool=2) [msb ... lsb]:"; show_format "Print format string?"; outputToWorkspace "Output to workspace?"; variablePrefix "Variable name prefix:"; outputToModelAsWell "Output to model as well?"
      mask help:
      | Expands a 'bus' made using a bus_create or Xilinx
      | concat block.
      | The input will be divided into the specified number
      | of outputs with the specified arithmetic types.
      | Divisions are made from most significant bit.
      mask init: same as s_b2a4x1kf/bus_expand
      settings: AttributesFormatString=12 outputs: uf32.0,uf32.0,uf32.0,uf32.0,uf32.0,uf32.0,uf32.0,uf32.0,uf32.0,uf32.0,uf32.0,uf32.0,
      mask TypeOptions mode: divisions of equal size | divisions of arbitrary size
      mask Callback mode: bus_expand_callback();
      mask Callback outputWidth: bus_expand_callback();
      mask Callback outputToWorkspace: bus_expand_callback();
  addsub{1..12} (12 alike) : xbsIndex_r4/AddSub  mode=Addition  use_carryin=off  use_carryout=off  en=off  latency=1  precision=User Defined  arith_type=Unsigned  n_bits=32  bin_pt=0  quantization=Truncate  overflow=Wrap  use_behavioral_HDL=on  hw_selection=Fabric  pipelined=on  dbl_ovrd=off  block_type=addsub
  b_debus : Subsystem  AncestorBlock=casper_library_flow_control/bus_expand  mask(bus_expand){mode=divisions of arbitrary size, outputNum=1, outputWidth=[3  3  3  3  3  3  3  3  3  3  3  3], outputBinaryPt=[0  0  0  0  0  0  0  0  0  0  0  0], outputArithmeticType=[0  0  0  0  0  0  0  0  0  0  0  0], show_format=on, outputToWorkspace=off, variablePrefix=, outputToModelAsWell=on}
      mask prompts: outputNum "Number of outputs:"; outputWidth "Output width [msb ... lsb]:"; outputBinaryPt "Output binary point position [msb ... lsb]:"; outputArithmeticType "Output arithmetic type (ufix=0, fix=1, bool=2) [msb ... lsb]:"; show_format "Print format string?"; outputToWorkspace "Output to workspace?"; variablePrefix "Variable name prefix:"; outputToModelAsWell "Output to model as well?"
      mask help:
      | Expands a 'bus' made using a bus_create or Xilinx
      | concat block.
      | The input will be divided into the specified number
      | of outputs with the specified arithmetic types.
      | Divisions are made from most significant bit.
      mask init: same as s_b2a4x1kf/bus_expand
      settings: AttributesFormatString=12 outputs: uf3.0,uf3.0,uf3.0,uf3.0,uf3.0,uf3.0,uf3.0,uf3.0,uf3.0,uf3.0,uf3.0,uf3.0,
      mask TypeOptions mode: divisions of equal size | divisions of arbitrary size
      mask Callback mode: bus_expand_callback();
      mask Callback outputWidth: bus_expand_callback();
      mask Callback outputToWorkspace: bus_expand_callback();
  op_bussify : Subsystem  AncestorBlock=casper_library_flow_control/bus_create  mask(bus_create){inputNum=12}
      mask prompts: inputNum "Number of inputs:"
      mask init:
      | bus_create_init(gcb,...
      |     'inputNum', inputNum);
  dout : Outport
  wires:
  a/1 -> a_debus/1(bus_in)
  b/1 -> b_debus/1(bus_in)
  a_debus/1(msb_out12) -> addsub1/1
  b_debus/1(msb_out12) -> addsub1/2
  a_debus/2(out11) -> addsub2/1
  b_debus/2(out11) -> addsub2/2
  a_debus/3(out10) -> addsub3/1
  b_debus/3(out10) -> addsub3/2
  a_debus/4(out9) -> addsub4/1
  b_debus/4(out9) -> addsub4/2
  a_debus/5(out8) -> addsub5/1
  b_debus/5(out8) -> addsub5/2
  a_debus/6(out7) -> addsub6/1
  b_debus/6(out7) -> addsub6/2
  a_debus/7(out6) -> addsub7/1
  b_debus/7(out6) -> addsub7/2
  a_debus/8(out5) -> addsub8/1
  b_debus/8(out5) -> addsub8/2
  a_debus/9(out4) -> addsub9/1
  b_debus/9(out4) -> addsub9/2
  a_debus/10(out3) -> addsub10/1
  b_debus/10(out3) -> addsub10/2
  a_debus/11(out2) -> addsub11/1
  b_debus/11(out2) -> addsub11/2
  a_debus/12(lsb_out1) -> addsub12/1
  b_debus/12(lsb_out1) -> addsub12/2
  addsub1/1 -> op_bussify/1(in1)
  addsub2/1 -> op_bussify/2(in2)
  addsub3/1 -> op_bussify/3(in3)
  addsub4/1 -> op_bussify/4(in4)
  addsub5/1 -> op_bussify/5(in5)
  addsub6/1 -> op_bussify/6(in6)
  addsub7/1 -> op_bussify/7(in7)
  addsub8/1 -> op_bussify/8(in8)
  addsub9/1 -> op_bussify/9(in9)
  addsub10/1 -> op_bussify/10(in10)
  addsub11/1 -> op_bussify/11(in11)
  addsub12/1 -> op_bussify/12(in12)
  op_bussify/1(bus_out) -> dout/1

== system s_b2a4x1kf/bus_expand ==
  bus_in : Inport
  reinterpret{1..12} (12 alike) : xbsIndex_r4/Reinterpret  force_arith_type=on  arith_type=Unsigned  force_bin_pt=on  bin_pt=0  block_type=reinterpret
  slice1 : xbsIndex_r4/Slice  nbits=32  boolean_output=off  mode=Upper Bit Location + Width  bit1=-352  base1=MSB of Input  bit0=0  base0=LSB of Input  dbl_ovrd=off  block_type=slice
  slice10 : xbsIndex_r4/Slice  nbits=32  boolean_output=off  mode=Upper Bit Location + Width  bit1=-64  base1=MSB of Input  bit0=0  base0=LSB of Input  dbl_ovrd=off  block_type=slice
  slice11 : xbsIndex_r4/Slice  nbits=32  boolean_output=off  mode=Upper Bit Location + Width  bit1=-32  base1=MSB of Input  bit0=0  base0=LSB of Input  dbl_ovrd=off  block_type=slice
  slice12 : xbsIndex_r4/Slice  nbits=32  boolean_output=off  mode=Upper Bit Location + Width  bit1=0  base1=MSB of Input  bit0=0  base0=LSB of Input  dbl_ovrd=off  block_type=slice
  slice2 : xbsIndex_r4/Slice  nbits=32  boolean_output=off  mode=Upper Bit Location + Width  bit1=-320  base1=MSB of Input  bit0=0  base0=LSB of Input  dbl_ovrd=off  block_type=slice
  slice3 : xbsIndex_r4/Slice  nbits=32  boolean_output=off  mode=Upper Bit Location + Width  bit1=-288  base1=MSB of Input  bit0=0  base0=LSB of Input  dbl_ovrd=off  block_type=slice
  slice4 : xbsIndex_r4/Slice  nbits=32  boolean_output=off  mode=Upper Bit Location + Width  bit1=-256  base1=MSB of Input  bit0=0  base0=LSB of Input  dbl_ovrd=off  block_type=slice
  slice5 : xbsIndex_r4/Slice  nbits=32  boolean_output=off  mode=Upper Bit Location + Width  bit1=-224  base1=MSB of Input  bit0=0  base0=LSB of Input  dbl_ovrd=off  block_type=slice
  slice6 : xbsIndex_r4/Slice  nbits=32  boolean_output=off  mode=Upper Bit Location + Width  bit1=-192  base1=MSB of Input  bit0=0  base0=LSB of Input  dbl_ovrd=off  block_type=slice
  slice7 : xbsIndex_r4/Slice  nbits=32  boolean_output=off  mode=Upper Bit Location + Width  bit1=-160  base1=MSB of Input  bit0=0  base0=LSB of Input  dbl_ovrd=off  block_type=slice
  slice8 : xbsIndex_r4/Slice  nbits=32  boolean_output=off  mode=Upper Bit Location + Width  bit1=-128  base1=MSB of Input  bit0=0  base0=LSB of Input  dbl_ovrd=off  block_type=slice
  slice9 : xbsIndex_r4/Slice  nbits=32  boolean_output=off  mode=Upper Bit Location + Width  bit1=-96  base1=MSB of Input  bit0=0  base0=LSB of Input  dbl_ovrd=off  block_type=slice
  msb_out12 : Outport
  out11 : Outport  Port=2
  out10 : Outport  Port=3
  out9 : Outport  Port=4
  out8 : Outport  Port=5
  out7 : Outport  Port=6
  out6 : Outport  Port=7
  out5 : Outport  Port=8
  out4 : Outport  Port=9
  out3 : Outport  Port=10
  out2 : Outport  Port=11
  lsb_out1 : Outport  Port=12
  wires:
  bus_in/1 -> slice12/1, slice11/1, slice10/1, slice9/1, slice8/1, slice7/1, slice6/1, slice5/1, slice4/1, slice3/1, slice2/1, slice1/1
  slice12/1 -> reinterpret12/1
  reinterpret12/1 -> msb_out12/1
  slice11/1 -> reinterpret11/1
  reinterpret11/1 -> out11/1
  slice10/1 -> reinterpret10/1
  reinterpret10/1 -> out10/1
  slice9/1 -> reinterpret9/1
  reinterpret9/1 -> out9/1
  slice8/1 -> reinterpret8/1
  reinterpret8/1 -> out8/1
  slice7/1 -> reinterpret7/1
  reinterpret7/1 -> out7/1
  slice6/1 -> reinterpret6/1
  reinterpret6/1 -> out6/1
  slice5/1 -> reinterpret5/1
  reinterpret5/1 -> out5/1
  slice4/1 -> reinterpret4/1
  reinterpret4/1 -> out4/1
  slice3/1 -> reinterpret3/1
  reinterpret3/1 -> out3/1
  slice2/1 -> reinterpret2/1
  reinterpret2/1 -> out2/1
  slice1/1 -> reinterpret1/1
  reinterpret1/1 -> lsb_out1/1

== system s_b2a4x1kf/bus_expand1 ==
  bus_in : Inport
  slice1 : xbsIndex_r4/Slice  nbits=1  boolean_output=on  mode=Upper Bit Location + Width  bit1=-11  base1=MSB of Input  bit0=0  base0=LSB of Input  dbl_ovrd=off  block_type=slice
  slice10 : xbsIndex_r4/Slice  nbits=1  boolean_output=on  mode=Upper Bit Location + Width  bit1=-2  base1=MSB of Input  bit0=0  base0=LSB of Input  dbl_ovrd=off  block_type=slice
  slice11 : xbsIndex_r4/Slice  nbits=1  boolean_output=on  mode=Upper Bit Location + Width  bit1=-1  base1=MSB of Input  bit0=0  base0=LSB of Input  dbl_ovrd=off  block_type=slice
  slice12 : xbsIndex_r4/Slice  nbits=1  boolean_output=on  mode=Upper Bit Location + Width  bit1=0  base1=MSB of Input  bit0=0  base0=LSB of Input  dbl_ovrd=off  block_type=slice
  slice2 : xbsIndex_r4/Slice  nbits=1  boolean_output=on  mode=Upper Bit Location + Width  bit1=-10  base1=MSB of Input  bit0=0  base0=LSB of Input  dbl_ovrd=off  block_type=slice
  slice3 : xbsIndex_r4/Slice  nbits=1  boolean_output=on  mode=Upper Bit Location + Width  bit1=-9  base1=MSB of Input  bit0=0  base0=LSB of Input  dbl_ovrd=off  block_type=slice
  slice4 : xbsIndex_r4/Slice  nbits=1  boolean_output=on  mode=Upper Bit Location + Width  bit1=-8  base1=MSB of Input  bit0=0  base0=LSB of Input  dbl_ovrd=off  block_type=slice
  slice5 : xbsIndex_r4/Slice  nbits=1  boolean_output=on  mode=Upper Bit Location + Width  bit1=-7  base1=MSB of Input  bit0=0  base0=LSB of Input  dbl_ovrd=off  block_type=slice
  slice6 : xbsIndex_r4/Slice  nbits=1  boolean_output=on  mode=Upper Bit Location + Width  bit1=-6  base1=MSB of Input  bit0=0  base0=LSB of Input  dbl_ovrd=off  block_type=slice
  slice7 : xbsIndex_r4/Slice  nbits=1  boolean_output=on  mode=Upper Bit Location + Width  bit1=-5  base1=MSB of Input  bit0=0  base0=LSB of Input  dbl_ovrd=off  block_type=slice
  slice8 : xbsIndex_r4/Slice  nbits=1  boolean_output=on  mode=Upper Bit Location + Width  bit1=-4  base1=MSB of Input  bit0=0  base0=LSB of Input  dbl_ovrd=off  block_type=slice
  slice9 : xbsIndex_r4/Slice  nbits=1  boolean_output=on  mode=Upper Bit Location + Width  bit1=-3  base1=MSB of Input  bit0=0  base0=LSB of Input  dbl_ovrd=off  block_type=slice
  msb_out12 : Outport
  out11 : Outport  Port=2
  out10 : Outport  Port=3
  out9 : Outport  Port=4
  out8 : Outport  Port=5
  out7 : Outport  Port=6
  out6 : Outport  Port=7
  out5 : Outport  Port=8
  out4 : Outport  Port=9
  out3 : Outport  Port=10
  out2 : Outport  Port=11
  lsb_out1 : Outport  Port=12
  wires:
  bus_in/1 -> slice12/1, slice11/1, slice10/1, slice9/1, slice8/1, slice7/1, slice6/1, slice5/1, slice4/1, slice3/1, slice2/1, slice1/1
  slice12/1 -> msb_out12/1
  slice11/1 -> out11/1
  slice10/1 -> out10/1
  slice9/1 -> out9/1
  slice8/1 -> out8/1
  slice7/1 -> out7/1
  slice6/1 -> out6/1
  slice5/1 -> out5/1
  slice4/1 -> out4/1
  slice3/1 -> out3/1
  slice2/1 -> out2/1
  slice1/1 -> lsb_out1/1
